simulink model "Lab4_p3_13b"  (R2013b)
settings: Solver=FixedStepDiscrete  SolverMode=SingleTasking  StartTime=0.0  StopTime=inf  FixedStep=.03  RelTol=1e-3
values from neighbouring files (symbols this model uses):
  cx = (xmax+xmin)/2    [MagAnalysis.m]
  cy = (ymax+ymin)/2    [MagAnalysis.m]
  dx = double(xmax-xmin)    [MagAnalysis.m]
  dy = double(ymax-ymin)    [MagAnalysis.m]
settings Model: SimulationMode=external  ExtModeTrigDuration=2  Creator=Alec  LastModifiedBy=nding
settings OptimizationCC: ExpressionDepthLimit=2147483647  OptimizeModelRefInitCode=on  LifeSpan=1
settings DebuggingCC: SolverPrmCheckMsg=none  StateNameClashWarn=warning
settings HardwareCC: ProdBitPerInt=16  ProdBitPerPointer=8  ProdIntDivRoundTo=Zero  ProdEndianess=LittleEndian  ProdWordSize=8  ProdHWDeviceType=Atmel->AVR
settings RTWCC: SystemTargetFile=realtime.tlc  GenerateMakefile=off  TemplateMakefile=realtime.tmf  Description=Real-Time Toolbox  RTWVerbose=off  ProcessScript=realtime_make_rtw_hook
settings CodeAppCC: CustomSymbolStrType=$N$R$M  InternalIdentifier=Classic
settings STFCustomTargetCC: TargetLibSuffix=.a  GenerateSampleERTMain=on  ERTCustomFileBanners=on  SupportNonInlinedSFcns=off  SupportVariableSizeSignals=on  MATLABClassNameForMDSCustomization=Simulink.SoftwareTarget.ERTCustomization  GRTInterface=off  SystemTargetFile=realtime.tlc
settings ERTTargetCC: CodeReplacementLibrary=ANSI_C  GenerateSampleERTMain=on  ParMdlRefBuildCompliant=off  CompOptLevelCompliant=off  ConcurrentExecutionCompliant=off  CombineOutputUpdateFcns=off  ERTFirstTimeCompliant=off  SupportContinuousTime=on  SupportVariableSizeSignals=on  ModelStepFunctionPrototypeControlCompliant=off  CPPClassGenCompliant=off  ExtMode=on  ExtModeTransport=3  ExtModeMexArgs=0 21 115200  InlinedParameterPlacement=NonHierarchical  ERTSrcFileBannerTemplate=realtime_code_template.cgt  ERTHdrFileBannerTemplate=realtime_code_template.cgt  ERTDataSrcFileTemplate=realtime_code_template.cgt  ERTDataHdrFileTemplate=realtime_code_template.cgt  ERTCustomFileTemplate=realtime_file_process.tlc

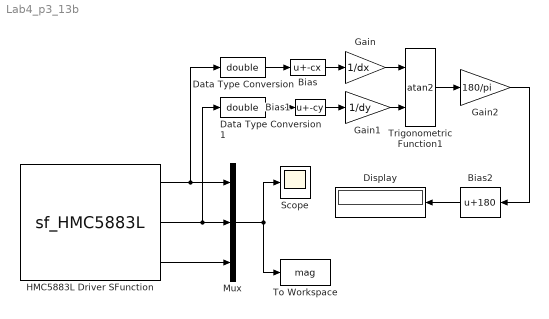
== system Lab4_p3_13b ==
  Bias : Bias  Bias=-cx
  Bias1 : Bias  Bias=-cy
  Bias2 : Bias  Bias=180
  Data Type Conversion : DataTypeConversion  OutDataTypeStr=double
  Data Type Conversion1 : DataTypeConversion  OutDataTypeStr=double
  Display : Display
  Gain : Gain  Gain=1/dx
  Gain1 : Gain  Gain=1/dy
  Gain2 : Gain  Gain=180/pi
  HMC5883L Driver SFunction : S-Function  InitFcn=try, set_param(gcb,'FunctionName','sf_HMC5883L'), end  FunctionName=sf_HMC5883L  SFunctionModules=sf_HMC5883L_wrapper  EnableBusSupport=off  mask(S-Function Builder){}
      mask help: Simulink:masks:SFunctionBuilder_MD
      mask init:
      | val = [[.9  0.75 0.75 1 1 .9 .9 1]',[1 1 0.75 0.75 .9 .9 1 .9]'];try , sys = get_param(gcb,'SfunBuilderFcnName');if isempty(sys), sys = get_param(gcb,'FunctionName'); end,catch, sys = get_param(gcb,'FunctionName'); end
      settings: CopyFcn=set_param(gcbh,'LinkStatus','none')  PreSaveFcn=try, set_param(gcb,'FunctionName','sf_HMC5883L'), end  OpenFcn=sfunctionwizard(gcbh)
      mask Display:
      | plot(val(:,1),val(:,2))
      | disp(sys)
      | port_label('output',1,'x_val')
      | port_label('output',2,'y_val')
      | port_label('output',3,'z_val')
  Mux : Mux  Inputs=3
  Scope : Scope
      settings: YMin=-300  YMax=250
  To Workspace : ToWorkspace  VariableName=mag  SampleTime=-1
  Trigonometric Function1 : Trigonometry  Operator=atan2
  wires:
  HMC5883L Driver SFunction/3 -> Mux/3
  Mux/1 -> To Workspace/1, Scope/1
  HMC5883L Driver SFunction/1 -> Data Type Conversion/1, Mux/1
  HMC5883L Driver SFunction/2 -> Data Type Conversion1/1, Mux/2
  Data Type Conversion/1 -> Bias/1
  Data Type Conversion1/1 -> Bias1/1
  Bias/1 -> Gain/1
  Bias1/1 -> Gain1/1
  Gain/1 -> Trigonometric Function1/1
  Gain1/1 -> Trigonometric Function1/2
  Trigonometric Function1/1 -> Gain2/1
  Gain2/1 -> Bias2/1
  Bias2/1 -> Display/1
